simulink subsystem "PowerSplitHEV_DirectInput_refsub"  (R2023a)
settings: Solver=VariableStepAuto  StartTime=0.0  StopTime=10.0  RelTol=1e-3
settings Model: Creator=isaacito  LastModifiedBy=isaacito
settings SolverCC: AlgebraicLoopSolver=TrustRegion
settings OptimizationCC: ReuseModelBlockBuffer=off
settings DebuggingCC: UnconnectedInputMsg=warning  UnconnectedOutputMsg=warning  UnconnectedLineMsg=warning
settings ModelReferenceCC: EnableRefExpFcnMdlSchedulingChecks=on
settings RTWCC: DLArmComputeVersion=19.05

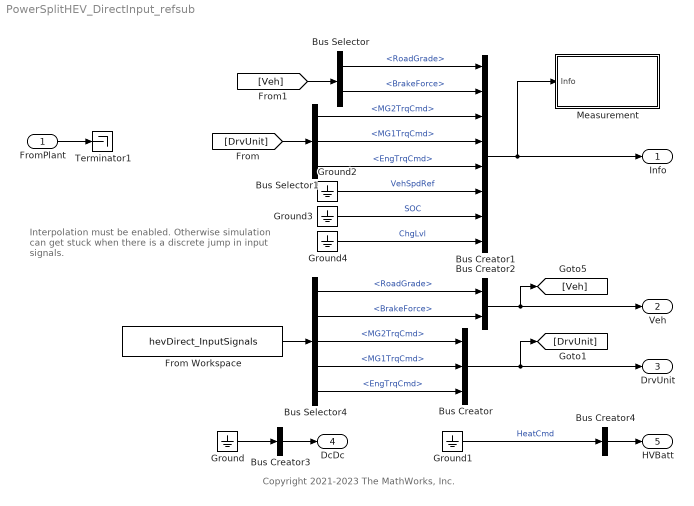
== system PowerSplitHEV_DirectInput_refsub ==
  note: Interpolation must be enabled.
      | Otherwise simulation can get stuck
      | when there is a discrete jump
      | in input signals.
  note: Copyright 2021-2023 The MathWorks, Inc.
  FromPlant : Inport
  Bus Creator : BusCreator  Inputs=3
  Bus Creator1 : BusCreator  Inputs=8
  Bus Creator2 : BusCreator  Inputs=2
  Bus Creator3 : BusCreator  Inputs=1
  Bus Creator4 : BusCreator  Inputs=1
  Bus Selector : BusSelector  OutputSignals=RoadGrade,BrakeForce
  Bus Selector1 : BusSelector  OutputSignals=MG2TrqCmd,MG1TrqCmd,EngTrqCmd
  Bus Selector4 : BusSelector  OutputSignals=RoadGrade,BrakeForce,MG2TrqCmd,MG1TrqCmd,EngTrqCmd
  From Workspace : FromWorkspace  VariableName=hevDirect_InputSignals  OutDataTypeStr=Bus: hevDirect_InputBus  OutputAfterFinalValue=Holding final value
      settings: AttributesFormatString=|
      | %<OutDataTypeStr>
      | Interpolate: %<Interpolate>
  Ground{,1..4} (5 alike) : Ground
  Measurement : Subsystem
  Terminator1 : Terminator
  Info : Outport
  Veh : Outport  Port=2
  DrvUnit : Outport  Port=3
  DcDc : Outport  Port=4
  HVBatt : Outport  Port=5
  wires:
  Bus Selector4/1 -> Bus Creator2/1  "<RoadGrade>"
  Bus Selector4/2 -> Bus Creator2/2  "<BrakeForce>"
  Bus Creator/1 -> [DrvUnit], DrvUnit/1
  Bus Selector4/3 -> Bus Creator/1  "<MG2TrqCmd>"
  Bus Selector4/4 -> Bus Creator/2  "<MG1TrqCmd>"
  Bus Selector4/5 -> Bus Creator/3  "<EngTrqCmd>"
  From Workspace/1 -> Bus Selector4/1
  Bus Creator1/1 -> Info/1, Measurement/1(Info)
  FromPlant/1 -> Terminator1/1
  Bus Creator2/1 -> Veh/1, [Veh]
  Ground1/1 -> Bus Creator4/1  "HeatCmd"
  Bus Creator4/1 -> HVBatt/1
  Bus Creator3/1 -> DcDc/1
  Ground/1 -> Bus Creator3/1
  Ground2/1 -> Bus Creator1/6  "VehSpdRef"
  Ground3/1 -> Bus Creator1/7  "SOC"
  [Veh] -> Bus Selector/1
  Bus Selector/1 -> Bus Creator1/1  "<RoadGrade>"
  Bus Selector/2 -> Bus Creator1/2  "<BrakeForce>"
  [DrvUnit] -> Bus Selector1/1
  Bus Selector1/1 -> Bus Creator1/3  "<MG2TrqCmd>"
  Bus Selector1/2 -> Bus Creator1/4  "<MG1TrqCmd>"
  Bus Selector1/3 -> Bus Creator1/5  "<EngTrqCmd>"
  Ground4/1 -> Bus Creator1/8  "ChgLvl"

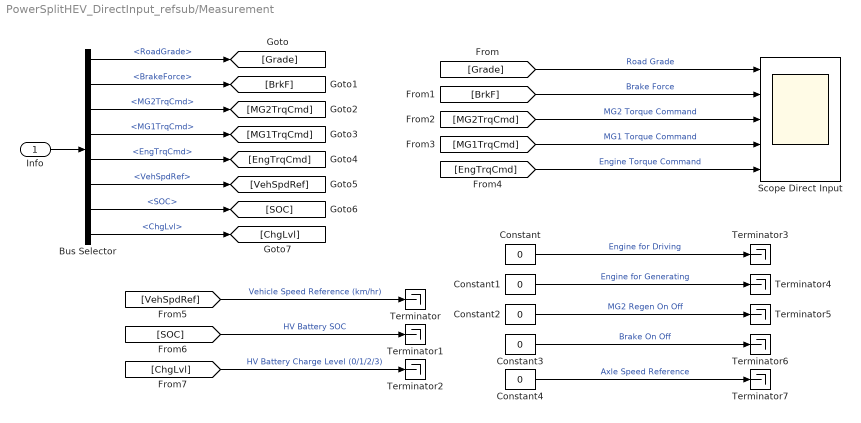
== system PowerSplitHEV_DirectInput_refsub/Measurement ==
  Info : Inport
  Bus Selector : BusSelector  OutputSignals=RoadGrade,BrakeForce,MG2TrqCmd,MG1TrqCmd,EngTrqCmd,VehSpdRef,SOC,ChgLvl
  Constant{,1..4} (5 alike) : Constant  Value=0
  Scope Direct Input : Scope  NumInputPorts=5
  Terminator{,1..7} (8 alike) : Terminator
  wires:
  [ChgLvl] -> Terminator2/1  "HV Battery Charge Level (0/1/2/3)"
  Bus Selector/8 -> [ChgLvl]  "<ChgLvl>"
  [SOC] -> Terminator1/1  "HV Battery SOC"
  [VehSpdRef] -> Terminator/1  "Vehicle Speed Reference (km/hr)"
  Bus Selector/6 -> [VehSpdRef]  "<VehSpdRef>"
  Bus Selector/7 -> [SOC]  "<SOC>"
  [EngTrqCmd] -> Scope Direct Input/5  "Engine Torque Command"
  [MG1TrqCmd] -> Scope Direct Input/4  "MG1 Torque Command"
  [MG2TrqCmd] -> Scope Direct Input/3  "MG2 Torque Command"
  [BrkF] -> Scope Direct Input/2  "Brake Force"
  [Grade] -> Scope Direct Input/1  "Road Grade"
  Bus Selector/2 -> [BrkF]  "<BrakeForce>"
  Bus Selector/3 -> [MG2TrqCmd]  "<MG2TrqCmd>"
  Bus Selector/4 -> [MG1TrqCmd]  "<MG1TrqCmd>"
  Bus Selector/5 -> [EngTrqCmd]  "<EngTrqCmd>"
  Bus Selector/1 -> [Grade]  "<RoadGrade>"
  Info/1 -> Bus Selector/1
  Constant1/1 -> Terminator4/1  "Engine for Generating"
  Constant/1 -> Terminator3/1  "Engine for Driving"
  Constant2/1 -> Terminator5/1  "MG2 Regen On Off"
  Constant3/1 -> Terminator6/1  "Brake On Off"
  Constant4/1 -> Terminator7/1  "Axle Speed Reference"
